simulink model "single_phase_ttype_inverter"  (R2026a)
settings: Solver=ode23tb  StopTime=simlength  FixedStep=tc  MaxStep=glb_time.tc
values from neighbouring files (symbols this model uses):
  afe_ctrl = param.afe.ctrl    [init_model.m]
  afe_pwm_phase_shift_mod1 = param.afe.behav.pwm_phase_shift_mod1    [init_model.m]
  DThs_init = param.thermal.DThs_init    [init_model.m]
  filters = param.ctrl.filters    [init_model.m]
  frt_data = param.frt.data    [init_model.m]
  glb_time = param.glb_time    [init_model.m]
  grid_emu = param.grid.emu    [init_model.m]
  kepsilon = param.spinv.kepsilon    [init_model.m]
  kp_align = param.ctrl.kp_align    [init_model.m]
  lim_down_align = param.ctrl.lim_down_align    [init_model.m]
  lim_up_align = param.ctrl.lim_up_align    [init_model.m]
  mavarage_filter_frequency_base_order = param.ctrl.mavarage_filter_frequency_base_order    [init_model.m]
  omega_set = param.spinv.omega_set    [init_model.m]
  single_phase_inverter_ctrl = param.spinv.ctrl    [init_model.m]
  Tambient = param.thermal.Tambient    [init_model.m]
  time_aux_power_supply_fault = param.sim.time_aux_power_supply_fault    [init_model.m]
  time_step_ref_1 = param.spinv.ref.time_step_ref_1    [init_model.m]
  time_step_ref_2 = param.spinv.ref.time_step_ref_2    [init_model.m]
  time_step_ref_3 = param.spinv.ref.time_step_ref_3    [init_model.m]
undefined symbols (not defined in the file or in its folder): delta_fht1, hwdata, ki_align, Ld_fht1, magnitude, omega_fht1, ts_inv, Vac_FS, Vdc_nom, Xbez
libraries: fl_lib x61, nesl_utility x39, moving_average_filter x11, moving_average_filter_cc x8, discrete_time_low_pass_filter x4, sl_discontinuities x3, single_phase_transformer_lib x3, linear_double_integrator_observer_ccaller x2, phase_shift_filter_ccaller x2, threephase_inductor_lib x1, dclink_for_two_levels x1, three_phase_pwm_modulator x1
(part 7 of 9)

== system single_phase_ttype_inverter/single_phase_inverter/single phase inverter control/single_phase_inverter_ctrl/phase generator/dq_pll_ccaller/first_harmonic_tracker3 ==
  u : Inport
  Bus Selector : BusSelector  OutputSignals=output_pu_hat
  Constant : Constant  Value=glb_time.ts_inv
  Constant1 : Constant  Value=4
  Constant2 : Constant  Value=afe_ctrl.fht_grid.omega_fht
  Constant3 : Constant  Value=afe_ctrl.fht_grid.delta_fht
  Constant4 : Constant  Value=afe_ctrl.fht_grid.Ld_fht(1)
  Constant5 : Constant  Value=afe_ctrl.fht_grid.Ld_fht(2)
  Data Type Conversion{1..2,6..9} (6 alike) : DataTypeConversion  OutDataTypeStr=single  SaturateOnIntegerOverflow=off  RndMeth=Floor
  Data Type Conversion3 : DataTypeConversion  OutDataTypeStr=uint8  SaturateOnIntegerOverflow=off  RndMeth=Floor
  Data Type Conversion4 : DataTypeConversion  OutDataTypeStr=double  SaturateOnIntegerOverflow=off  RndMeth=Floor
  Data Type Conversion5 : DataTypeConversion  OutDataTypeStr=uint8  SaturateOnIntegerOverflow=off  RndMeth=Floor
  Step : Step  Time=0.0125  InitialValue=1  FinalValue=0
  first_harmonic_tracker : CCaller  FunctionName=first_harmonic_tracker_process_simulink  PortSpecificationStruct="%)30     .    B \\   8    (     @         %    \"     D    !     0         %  0 \"0    $    _    07)G3F%M90  4&]R=$YA;64 4V-O<&4     26YD97@     5'EP90      4VEZ90      27-';&]B86P   X    P    !@    @    $          4    (     0    ,    !         !   P!O=70 #@   #     &    \"     0         !0    @    !     P    $         $  # &]U=  .    .     8    (    !          %    \"     $    &     0         0  ...(+4988 chars)"
  u_hat : Outport
  wires:
  Data Type Conversion4/1 -> u_hat/1
  Data Type Conversion3/1 -> first_harmonic_tracker/1
  Data Type Conversion1/1 -> first_harmonic_tracker/3
  Data Type Conversion2/1 -> first_harmonic_tracker/2
  first_harmonic_tracker/1 -> Bus Selector/1
  Bus Selector/1 -> Data Type Conversion4/1  "<output_pu_hat>"
  Step/1 -> Data Type Conversion3/1
  u/1 -> Data Type Conversion2/1
  Constant/1 -> Data Type Conversion1/1
  Constant1/1 -> Data Type Conversion5/1
  Data Type Conversion5/1 -> first_harmonic_tracker/8
  Constant2/1 -> Data Type Conversion6/1
  Data Type Conversion6/1 -> first_harmonic_tracker/4
  Constant3/1 -> Data Type Conversion7/1
  Data Type Conversion7/1 -> first_harmonic_tracker/5
  Constant4/1 -> Data Type Conversion8/1
  Data Type Conversion8/1 -> first_harmonic_tracker/6
  Constant5/1 -> Data Type Conversion9/1
  Data Type Conversion9/1 -> first_harmonic_tracker/7

== system single_phase_ttype_inverter/single_phase_inverter/single phase inverter control/single_phase_inverter_ctrl/phase_compensation_1/alignment_eval_afe1/pi ==
  u_ref : Inport
  u : Inport  Port=2
  1/Ti : Gain  Gain=kp  SaturateOnIntegerOverflow=on  OutDataTypeStr=Inherit: Same as input  ParamDataTypeStr=Inherit: Same as input
  Saturation : Saturate  UpperLimit=lim_up  LowerLimit=lim_down
  Sum1 : Sum  Inputs=+++  SaturateOnIntegerOverflow=on
  Sum2 : Sum  Inputs=-+  SaturateOnIntegerOverflow=on
  Sum3 : Sum  Inputs=-+  SaturateOnIntegerOverflow=on
  Unit Delay4 : UnitDelay  SampleTime=-1
  kp : Gain  Gain=ki  SaturateOnIntegerOverflow=on  OutDataTypeStr=Inherit: Same as input  ParamDataTypeStr=Inherit: Same as input
  y : Outport
  wires:
  1/Ti/1 -> Sum1/1, Sum3/1
  kp/1 -> Sum1/2
  Sum3/1 -> Unit Delay4/1
  Unit Delay4/1 -> Sum1/3
  u_ref/1 -> Sum2/2
  u/1 -> Sum2/1
  Sum2/1 -> kp/1, 1/Ti/1
  Sum1/1 -> Saturation/1
  Saturation/1 -> Sum3/2, y/1

== system single_phase_ttype_inverter/single_phase_inverter/single phase inverter control/single_phase_inverter_ctrl/single_phase_current_control/dqpi_current_controller/alphabeta2dq ==
  alpha : Inport
  beta : Inport  Port=2
  MATLAB Function : MATLAB Function  TreatAsAtomicUnit=on
  "d " : Outport  VectorParamsAs1DForOutWhenUnconnected=off
  "q " : Outport  Port=2  VectorParamsAs1DForOutWhenUnconnected=off
  wires:
  alpha/1 -> MATLAB Function/1(alpha)
  beta/1 -> MATLAB Function/2(beta)
  MATLAB Function/1(d) -> "d "/1
  MATLAB Function/2(q) -> "q "/1
  [phase] -> MATLAB Function/3(phase)

== system single_phase_ttype_inverter/single_phase_inverter/single phase inverter control/single_phase_inverter_ctrl/single_phase_current_control/dqpi_current_controller/dq2alphabeta ==
  d : Inport
  q : Inport  Port=2
  MATLAB Function : MATLAB Function  TreatAsAtomicUnit=on
  alpha : Outport  VectorParamsAs1DForOutWhenUnconnected=off
  wires:
  d/1 -> MATLAB Function/1(d)
  q/1 -> MATLAB Function/2(q)
  MATLAB Function/1(alpha) -> alpha/1
  [phase] -> MATLAB Function/3(phase)

== system single_phase_ttype_inverter/single_phase_inverter/single phase inverter control/single_phase_inverter_ctrl/single_phase_current_control/dqpi_current_controller/dq_vector_pi ==
  id_ref : Inport
  id : Inport  Port=2
  iq : Inport  Port=3
  iq_ref : Inport  Port=4
  dq_vector_pi : dq_vector_pi/dq_vector_pi  kp=single_phase_inverter_ctrl.kp_inv  ki=single_phase_inverter_ctrl.ki_inv  ts=glb_time.ts_inv  lim_ctrl_out=1  CTRPIFF_CLIP_RELEASE=1e-3
  ud_ctrl : Outport
  uq_ctrl : Outport  Port=2
  wires:
  id_ref/1 -> dq_vector_pi/1  "id_ref"
  iq_ref/1 -> dq_vector_pi/3  "iq_ref"
  dq_vector_pi/1 -> ud_ctrl/1  "ud_ctrl"
  iq/1 -> dq_vector_pi/4  "iq"
  id/1 -> dq_vector_pi/2  "id"
  dq_vector_pi/2 -> uq_ctrl/1  "uq_ctrl"
  [dclink_voltage_pu] -> dq_vector_pi/5

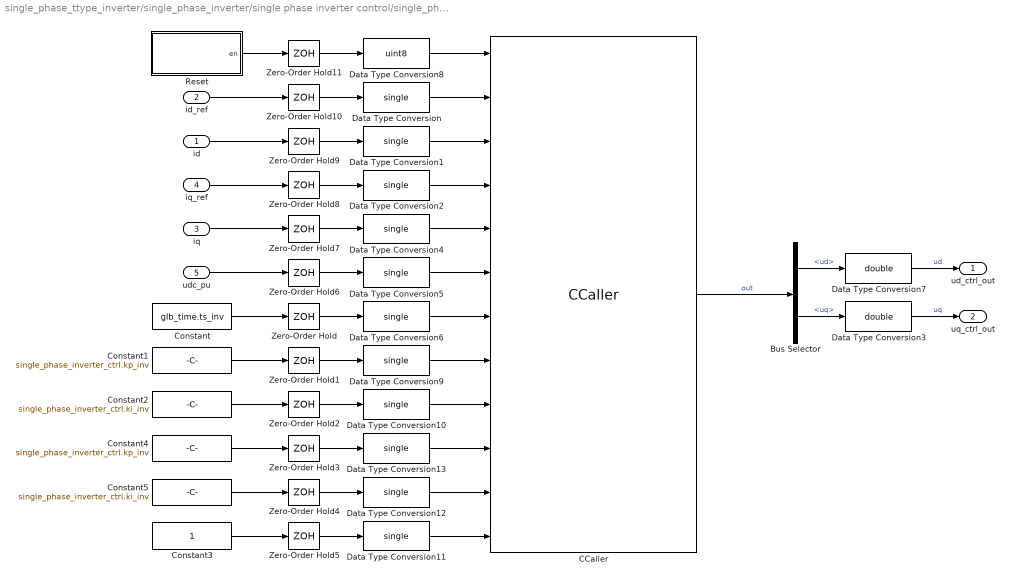
== system single_phase_ttype_inverter/single_phase_inverter/single phase inverter control/single_phase_inverter_ctrl/single_phase_current_control/dqpi_current_controller/dq_vector_pi_ccaller ==
  id : Inport
  id_ref : Inport  Port=2
  iq : Inport  Port=3
  iq_ref : Inport  Port=4
  udc_pu : Inport  Port=5
  Bus Selector : BusSelector  OutputSignals=ud,uq
  CCaller : CCaller  FunctionName=dqvector_pi_process_simulink  PortSpecificationStruct="%)30     .    ,!8   8    (     @         %    \"     T    !     0         %  0 \"0    $    _    07)G3F%M90  4&]R=$YA;64 4V-O<&4     26YD97@     5'EP90      4VEZ90      27-';&]B86P   X    P    !@    @    $          4    (     0    ,    !         !   P!O=70 #@   #     &    \"     0         !0    @    !     P    $         $  # &]U=  .    .     8    (    !          %    \"     $    &     0         0   ...(+7280 chars)"
  Constant : Constant  Value=glb_time.ts_inv
  Constant1 : Constant  Value=single_phase_inverter_ctrl.kp_inv
  Constant2 : Constant  Value=single_phase_inverter_ctrl.ki_inv
  Constant3 : Constant
  Constant4 : Constant  Value=single_phase_inverter_ctrl.kp_inv
  Constant5 : Constant  Value=single_phase_inverter_ctrl.ki_inv
  Data Type Conversion{,1..2,4..6,9..13} (11 alike) : DataTypeConversion  OutDataTypeStr=single  SaturateOnIntegerOverflow=off  RndMeth=Floor
  Data Type Conversion3 : DataTypeConversion  OutDataTypeStr=double  SaturateOnIntegerOverflow=off  RndMeth=Floor
  Data Type Conversion7 : DataTypeConversion  OutDataTypeStr=double  SaturateOnIntegerOverflow=off  RndMeth=Floor
  Data Type Conversion8 : DataTypeConversion  OutDataTypeStr=uint8  SaturateOnIntegerOverflow=off  RndMeth=Floor
  Reset : Subsystem
  Zero-Order Hold{,1..11} (12 alike) : ZeroOrderHold  SampleTime=-1
  ud_ctrl_out : Outport
  uq_ctrl_out : Outport  Port=2
  wires:
  Data Type Conversion5/1 -> CCaller/6
  Data Type Conversion/1 -> CCaller/2
  CCaller/1 -> Bus Selector/1  "out"
  Data Type Conversion1/1 -> CCaller/3
  Data Type Conversion4/1 -> CCaller/5
  Data Type Conversion2/1 -> CCaller/4
  Data Type Conversion6/1 -> CCaller/7
  Bus Selector/2 -> Data Type Conversion3/1  "<uq>"
  Bus Selector/1 -> Data Type Conversion7/1  "<ud>"
  Data Type Conversion7/1 -> ud_ctrl_out/1  "ud"
  Data Type Conversion3/1 -> uq_ctrl_out/1  "uq"
  Data Type Conversion8/1 -> CCaller/1
  Data Type Conversion9/1 -> CCaller/8
  Data Type Conversion10/1 -> CCaller/9
  Data Type Conversion11/1 -> CCaller/12
  Data Type Conversion13/1 -> CCaller/10
  Data Type Conversion12/1 -> CCaller/11
  Constant3/1 -> Zero-Order Hold5/1
  Constant5/1 -> Zero-Order Hold4/1
  Constant4/1 -> Zero-Order Hold3/1
  Constant2/1 -> Zero-Order Hold2/1
  Constant1/1 -> Zero-Order Hold1/1
  Constant/1 -> Zero-Order Hold/1
  udc_pu/1 -> Zero-Order Hold6/1
  iq/1 -> Zero-Order Hold7/1
  iq_ref/1 -> Zero-Order Hold8/1
  Reset/1(en) -> Zero-Order Hold11/1
  id_ref/1 -> Zero-Order Hold10/1
  id/1 -> Zero-Order Hold9/1
  Zero-Order Hold/1 -> Data Type Conversion6/1
  Zero-Order Hold1/1 -> Data Type Conversion9/1
  Zero-Order Hold2/1 -> Data Type Conversion10/1
  Zero-Order Hold3/1 -> Data Type Conversion13/1
  Zero-Order Hold4/1 -> Data Type Conversion12/1
  Zero-Order Hold5/1 -> Data Type Conversion11/1
  Zero-Order Hold6/1 -> Data Type Conversion5/1
  Zero-Order Hold7/1 -> Data Type Conversion4/1
  Zero-Order Hold8/1 -> Data Type Conversion2/1
  Zero-Order Hold9/1 -> Data Type Conversion1/1
  Zero-Order Hold10/1 -> Data Type Conversion/1
  Zero-Order Hold11/1 -> Data Type Conversion8/1

== system single_phase_ttype_inverter/single_phase_inverter/single phase inverter control/single_phase_inverter_ctrl/single_phase_current_control/dqpi_current_controller/i2alphabeta ==
  i_alpha : Inport
  Variant Source2 : VariantSource  VariantControls="{use_single_phase_inverter_based_FHT == 1, use_single_phase_inverter_based_SOGI  == 1, use_single_phase_inverter_based_PHSH  == 1, use_single_phase_inverter_based_SOGI_ccaller  == 1, use_single_phase_inverter_based_PHSH_ccaller  == 1}"
  Variant Source3 : VariantSource  VariantControls="{use_single_phase_inverter_based_FHT == 1, use_single_phase_inverter_based_SOGI  == 1, use_single_phase_inverter_based_PHSH  == 1, use_single_phase_inverter_based_SOGI_ccaller  == 1, use_single_phase_inverter_based_PHSH_ccaller  == 1}"
  first_harmonic_tracker : Subsystem
  phase_shift_method : Subsystem
  phase_shift_method_ccaller : Subsystem
  sogi : Subsystem
  sogi_ccaller : Subsystem
  i_alpha_out : Outport
  i_beta_out : Outport  Port=2
  wires:
  i_alpha/1 -> phase_shift_method_ccaller/1(i_alpha), sogi_ccaller/1(input), phase_shift_method/1(i_alpha), sogi/1(u), first_harmonic_tracker/1(u)
  [i_alpha_phsh] -> Variant Source2/3
  [i_beta_sogi] -> Variant Source3/2
  [i_alpha_phsh_cc] -> Variant Source2/5
  first_harmonic_tracker/2(beta) -> [i_beta_fht]  "i_beta_fht"
  phase_shift_method/2(i_beta_phase_shift_m) -> [i_beta_phsh]  "i_beta_phsh"
  phase_shift_method/1(i_alpha_phase_shift_m) -> [i_alpha_phsh]  "i_alpha_phsh"
  [i_alpha_sogi] -> Variant Source2/2
  phase_shift_method_ccaller/1(i_alpha_phase_shift_m) -> [i_alpha_phsh_cc]  "i_alpha_phsh_cc"
  [i_beta_phsh_cc] -> Variant Source3/5
  [i_alpha_fht] -> Variant Source2/1
  [i_beta_phsh] -> Variant Source3/3
  sogi_ccaller/1(alpha) -> [i_alpha_sogi_cc]  "i_alpha_sogi_cc"
  [i_beta_sogi_cc] -> Variant Source3/4
  sogi/1(ualpha) -> [i_alpha_sogi]  "i_alpha_sogi"
  sogi/2(ubeta) -> [i_beta_sogi]  "i_beta_sogi"
  phase_shift_method_ccaller/2(i_beta_phase_shift_m) -> [i_beta_phsh_cc]  "i_beta_phsh_cc"
  sogi_ccaller/2(beta) -> [i_beta_sogi_cc]  "i_beta_sogi_cc"
  Variant Source2/1 -> i_alpha_out/1  "i_alpha"
  first_harmonic_tracker/1(alpha) -> [i_alpha_fht]  "i_alpha_fht"
  [i_alpha_sogi_cc] -> Variant Source2/4
  [i_beta_fht] -> Variant Source3/1
  Variant Source3/1 -> i_beta_out/1  "i_beta"

== system single_phase_ttype_inverter/single_phase_inverter/single phase inverter control/single_phase_inverter_ctrl/single_phase_current_control/rpi_current_controller/Reset ==
  Step : Step  Time=0.05  InitialValue=1  FinalValue=0
  en : Outport
  wires:
  Step/1 -> en/1

== system single_phase_ttype_inverter/single_phase_inverter/single phase inverter control/single_phase_inverter_ctrl/sistem_identification/open loop u//f/dq2alphabeta ==
  Constant1 : Constant  Value=0
  Data Store Read : DataStoreRead  DataStoreName=u_test  IndexOptions=Index vector (dialog)  Indices=1  OutputSizes=1
  MATLAB Function : MATLAB Function  TreatAsAtomicUnit=on
  alpha : Outport  VectorParamsAs1DForOutWhenUnconnected=off
  wires:
  [phase] -> MATLAB Function/3(phase)
  MATLAB Function/1(alpha) -> alpha/1
  Data Store Read/1 -> MATLAB Function/1(d)
  Constant1/1 -> MATLAB Function/2(q)

== system single_phase_ttype_inverter/single_phase_inverter/single phase inverter control/single_phase_inverter_ctrl/sistem_identification/open loop u//f/first_harmonic_tracker ==
  u : Inport
  Bus Selector : BusSelector  OutputSignals=output_pu_hat,output_pu_hat_dot
  Constant : Constant  Value=ts_inv
  Constant1 : Constant  Value=8
  Constant2 : Constant  Value=omega_fht1
  Constant3 : Constant  Value=delta_fht1
  Constant4 : Constant  Value=Ld_fht1(1)
  Constant5 : Constant  Value=Ld_fht1(2)
  Data Type Conversion{1..2,6..9} (6 alike) : DataTypeConversion  OutDataTypeStr=single  SaturateOnIntegerOverflow=off  RndMeth=Floor
  Data Type Conversion10 : DataTypeConversion  OutDataTypeStr=double  SaturateOnIntegerOverflow=off  RndMeth=Floor
  Data Type Conversion3 : DataTypeConversion  OutDataTypeStr=uint8  SaturateOnIntegerOverflow=off  RndMeth=Floor
  Data Type Conversion4 : DataTypeConversion  OutDataTypeStr=double  SaturateOnIntegerOverflow=off  RndMeth=Floor
  Data Type Conversion5 : DataTypeConversion  OutDataTypeStr=uint8  SaturateOnIntegerOverflow=off  RndMeth=Floor
  Gain : Gain  Gain=-1/omega_fht1
  Step : Step  Time=0.0125  InitialValue=1  FinalValue=0
  first_harmonic_tracker : CCaller  FunctionName=first_harmonic_tracker_process_simulink  PortSpecificationStruct="%)30     .    B \\   8    (     @         %    \"     D    !     0         %  0 \"0    $    _    07)G3F%M90  4&]R=$YA;64 4V-O<&4     26YD97@     5'EP90      4VEZ90      27-';&]B86P   X    P    !@    @    $          4    (     0    ,    !         !   P!O=70 #@   #     &    \"     0         !0    @    !     P    $         $  # &]U=  .    .     8    (    !          %    \"     $    &     0         0  ...(+4988 chars)"
  alpha : Outport
  beta : Outport  Port=2
  wires:
  Data Type Conversion4/1 -> alpha/1
  Data Type Conversion3/1 -> first_harmonic_tracker/1
  Data Type Conversion1/1 -> first_harmonic_tracker/3
  Data Type Conversion2/1 -> first_harmonic_tracker/2
  first_harmonic_tracker/1 -> Bus Selector/1
  Bus Selector/1 -> Data Type Conversion4/1  "<output_pu_hat>"
  Step/1 -> Data Type Conversion3/1
  u/1 -> Data Type Conversion2/1
  Constant/1 -> Data Type Conversion1/1
  Constant1/1 -> Data Type Conversion5/1
  Data Type Conversion5/1 -> first_harmonic_tracker/8
  Constant2/1 -> Data Type Conversion6/1
  Data Type Conversion6/1 -> first_harmonic_tracker/4
  Constant3/1 -> Data Type Conversion7/1
  Data Type Conversion7/1 -> first_harmonic_tracker/5
  Constant4/1 -> Data Type Conversion8/1
  Data Type Conversion8/1 -> first_harmonic_tracker/6
  Constant5/1 -> Data Type Conversion9/1
  Data Type Conversion9/1 -> first_harmonic_tracker/7
  Bus Selector/2 -> Data Type Conversion10/1  "<output_pu_hat_dot>"
  Data Type Conversion10/1 -> Gain/1
  Gain/1 -> beta/1

== system single_phase_ttype_inverter/single_phase_inverter/single phase inverter control/single_phase_inverter_ctrl/sistem_identification/open loop u//f/module ==
  i_alpha : Inport
  i_beta : Inport  Port=2
  Sqrt : Sqrt
  Square : Math  Operator=square
  Square1 : Math  Operator=square
  Sum : Sum  Inputs=|++
  i : Outport
  wires:
  i_beta/1 -> Square1/1
  i_alpha/1 -> Square/1
  Square/1 -> Sum/1
  Sum/1 -> Sqrt/1
  Square1/1 -> Sum/2
  Sqrt/1 -> i/1  "i"

== system single_phase_ttype_inverter/single_phase_inverter/single phase inverter control/single_phase_inverter_ctrl/sistem_identification/open loop u//f/sogi_ccaller ==
  input : Inport
  Bus Selector : BusSelector  OutputSignals=sogi_flt_output_alpha,sogi_flt_output_beta
  CCaller : CCaller  FunctionName=sogi_flt_process_simulink  PortSpecificationStruct="%)30     .    . P   8    (     @         %    \"     <    !     0         %  0 \"0    $    _    07)G3F%M90  4&]R=$YA;64 4V-O<&4     26YD97@     5'EP90      4VEZ90      27-';&]B86P   X    P    !@    @    $          4    (     0    ,    !         !   P!O=70 #@   #     &    \"     0         !0    @    !     P    $         $  # &]U=  .    .     8    (    !          %    \"     $    &     0         0   ...(+3829 chars)"
  Constant1 : Constant  Value=ts_inv
  Constant2 : Constant  Value=omega_set
  Constant3 : Constant  Value=kepsilon
  Constant4 : Constant  Value=0
  Data Type Conversion{1..2,4,6} (4 alike) : DataTypeConversion  OutDataTypeStr=single  SaturateOnIntegerOverflow=off  RndMeth=Floor
  Data Type Conversion3 : DataTypeConversion  OutDataTypeStr=uint8  SaturateOnIntegerOverflow=off  RndMeth=Floor
  Data Type Conversion5 : DataTypeConversion  OutDataTypeStr=double  SaturateOnIntegerOverflow=off  RndMeth=Floor
  Data Type Conversion7 : DataTypeConversion  OutDataTypeStr=double  SaturateOnIntegerOverflow=off  RndMeth=Floor
  Data Type Conversion8 : DataTypeConversion  OutDataTypeStr=uint8  SaturateOnIntegerOverflow=off  RndMeth=Floor
  Reset : Subsystem
  Zero-Order Hold{1..6} (6 alike) : ZeroOrderHold  SampleTime=-1
  alpha : Outport
  beta : Outport  Port=2
  wires:
  Zero-Order Hold6/1 -> Data Type Conversion4/1
  Data Type Conversion7/1 -> alpha/1
  Data Type Conversion4/1 -> CCaller/1
  Bus Selector/1 -> Data Type Conversion7/1  "<sogi_flt_output_alpha>"
  CCaller/1 -> Bus Selector/1
  Constant4/1 -> Zero-Order Hold5/1
  Zero-Order Hold5/1 -> Data Type Conversion3/1
  Constant2/1 -> Zero-Order Hold1/1
  Zero-Order Hold1/1 -> Data Type Conversion2/1
  Zero-Order Hold2/1 -> Data Type Conversion1/1
  Constant1/1 -> Zero-Order Hold2/1
  Reset/1(en) -> Zero-Order Hold4/1
  Zero-Order Hold4/1 -> Data Type Conversion8/1
  input/1 -> Zero-Order Hold6/1
  Bus Selector/2 -> Data Type Conversion5/1  "<sogi_flt_output_beta>"
  Data Type Conversion5/1 -> beta/1
  Data Type Conversion3/1 -> CCaller/6
  Data Type Conversion8/1 -> CCaller/5
  Data Type Conversion2/1 -> CCaller/3
  Data Type Conversion1/1 -> CCaller/2
  Data Type Conversion6/1 -> CCaller/4
  Zero-Order Hold3/1 -> Data Type Conversion6/1
  Constant3/1 -> Zero-Order Hold3/1

== system single_phase_ttype_inverter/afe/AFE_control/afe_control/current_ctrl/inner_current_ctrl/anti_wind_up_ff/anti_wind_up ==
  alpha : Inport
  beta : Inport  Port=2
  Saturation : Saturate  UpperLimit=10  LowerLimit=1
  Sqrt : Sqrt
  Square : Math  Operator=square
  Square1 : Math  Operator=square
  Sum : Sum  Inputs=|++
  scaling : Outport
  wires:
  alpha/1 -> Square/1
  Sum/1 -> Sqrt/1
  beta/1 -> Square1/1
  Square/1 -> Sum/1
  Square1/1 -> Sum/2
  Sqrt/1 -> Saturation/1
  Saturation/1 -> scaling/1

== system single_phase_ttype_inverter/afe/AFE_control/afe_control/grid_voltage_phase_lock_loops/DDSRF-PLL/pll_stageA/filter_and_transformation ==
  ug_a : Inport
  ug_b : Inport  Port=2
  ug_c : Inport  Port=3
  abc2alphabeta : MATLAB Function  TreatAsAtomicUnit=on
  first_harmonic_tracker : Scope  NumInputPorts=3
      settings: ActiveDisplayYMinimum=-1.2482939809560776  ActiveDisplayYMaximum=1.2484282106161118  DataLoggingVariableName=ScopeData3
  first_harmonic_tracker_phase_u : Subsystem
  first_harmonic_tracker_phase_v : Subsystem
  first_harmonic_tracker_phase_w : Subsystem
  ug_alpha : Outport  VectorParamsAs1DForOutWhenUnconnected=off
  ug_beta : Outport  Port=2  VectorParamsAs1DForOutWhenUnconnected=off
  wires:
  abc2alphabeta/1(alpha) -> ug_alpha/1  "u_grid_alpha"
  abc2alphabeta/2(beta) -> ug_beta/1  "u_grid_beta"
  first_harmonic_tracker_phase_u/1(u_hat) -> first_harmonic_tracker/1, abc2alphabeta/1(a)  "tracker_phase_u"
  first_harmonic_tracker_phase_w/1(u_hat) -> first_harmonic_tracker/3, abc2alphabeta/3(c)  "tracker_phase_w"
  first_harmonic_tracker_phase_v/1(u_hat) -> first_harmonic_tracker/2, abc2alphabeta/2(b)  "tracker_phase_v"
  ug_a/1 -> first_harmonic_tracker_phase_u/1(u)
  ug_b/1 -> first_harmonic_tracker_phase_v/1(u)
  ug_c/1 -> first_harmonic_tracker_phase_w/1(u)

== system single_phase_ttype_inverter/afe/AFE_control/afe_control/grid_voltage_phase_lock_loops/DDSRF-PLL/pll_stageA/sequences ==
  u_grid_alpha : Inport
  u_grid_beta : Inport  Port=2
  phase_angle : Inport  Port=3
  ddsrf : Subsystem
  u_grid_pos_xi : Outport
  u_grid_pos_eta : Outport  Port=2
  wires:
  phase_angle/1 -> ddsrf/3(phase_angle)  "phase_angle"
  u_grid_beta/1 -> ddsrf/2(u_grid_beta)  "u_grid_beta"
  u_grid_alpha/1 -> ddsrf/1(u_grid_alpha)  "u_grid_alpha"
  ddsrf/4(u_grid_neg_eta) -> u_grid_pos_eta/1  "u_grid_pos_eta"
  ddsrf/3(u_grid_neg_xi) -> u_grid_pos_xi/1  "u_grid_pos_xi"

== system single_phase_ttype_inverter/afe/AFE_control/afe_control/grid_voltage_phase_lock_loops/DDSRF-PLL/pll_stageB/double_integrator_observer ==
  phase : Inport
  Gain : Gain  Gain=afe_ctrl.di_obs.Ldso  Multiplication=Matrix(K*u)
  Gain1 : Gain  Gain=afe_ctrl.di_obs.Adso  Multiplication=Matrix(K*u)
  Gain2 : Gain  Gain=afe_ctrl.di_obs.Cso  Multiplication=Matrix(K*u)
  Selector : Selector  InputPortWidth=2  IndexOptions=Index vector (dialog)  Indices=2  OutputSizes=1
  Sum : Sum  Inputs=-+|
  Sum1 : Sum  Inputs=|++
  Unit Delay : UnitDelay  SampleTime=-1
  bounder1 : MATLAB Function  TreatAsAtomicUnit=on
  bounder2 : MATLAB Function  TreatAsAtomicUnit=on
  omega_hat : Outport
  wires:
  Gain/1 -> Sum1/1
  Selector/1 -> omega_hat/1
  Gain2/1 -> bounder2/1(u)  "theta_hat"
  Gain1/1 -> Sum1/2
  Sum1/1 -> Unit Delay/1
  Sum/1 -> bounder1/1(u)  "e"
  Unit Delay/1 -> Gain1/1, Selector/1, Gain2/1
  phase/1 -> Sum/2  "phase"
  bounder1/1(y) -> Gain/1  "e_bounded"
  bounder2/1(y) -> Sum/1  "theta_hat_bounded"

== system single_phase_ttype_inverter/afe/AFE_control/afe_control/grid_voltage_phase_lock_loops/FHT-PLL/pll_stageA/filter_and_transformation ==
  ug_a : Inport
  ug_b : Inport  Port=2
  ug_c : Inport  Port=3
  Bus Creator : BusCreator  Inputs=2
  Bus Creator1 : BusCreator  Inputs=3
  Bus Creator2 : BusCreator  Inputs=2
  Bus Creator3 : BusCreator  Inputs=3
  Bus Creator4 : BusCreator  Inputs=3
  FHTalpha : Subsystem
  FHTbeta : Subsystem
  FHTdqPLL : Scope  NumInputPorts=2
      settings: ActiveDisplayYMinimum=-1.5258214459194912  ActiveDisplayYMaximum=1.5258228058860459  DataLoggingVariableName=ScopeData12
  Gain : Gain  Gain=-1/2
  Gain1 : Gain  Gain=-1/2
  Sum : Sum  Inputs=|++
  Sum1 : Sum  Inputs=-+|
  To Workspace1 : ToWorkspace  VariableName=ugd_alpha_sim  SampleTime=-1
      settings: MaxDataPoints=glb_time.Ns_afe
  To Workspace2 : ToWorkspace  VariableName=ugd_beta_sim  SampleTime=-1
      settings: MaxDataPoints=glb_time.Ns_afe
  To Workspace3 : ToWorkspace  VariableName=u_fht_alpha_sim  SampleTime=-1
      settings: MaxDataPoints=glb_time.Ns_afe
  To Workspace4 : ToWorkspace  VariableName=v_fht_alpha_sim  SampleTime=-1
      settings: MaxDataPoints=glb_time.Ns_afe
  To Workspace5 : ToWorkspace  VariableName=u_fhtsr_alpha_sim  SampleTime=-1
      settings: MaxDataPoints=glb_time.Ns_afe
  To Workspace6 : ToWorkspace  VariableName=u_fhtsr_beta_sim  SampleTime=-1
      settings: MaxDataPoints=glb_time.Ns_afe
  To Workspace7 : ToWorkspace  VariableName=u_fht_beta_sim  SampleTime=-1
      settings: MaxDataPoints=glb_time.Ns_afe
  To Workspace8 : ToWorkspace  VariableName=v_fht_beta_sim  SampleTime=-1
      settings: MaxDataPoints=glb_time.Ns_afe
  To Workspace9 : ToWorkspace  VariableName=ugd_abc_grid_sim  SampleTime=-1
      settings: MaxDataPoints=glb_time.Ns_afe
  abc2alphabeta : MATLAB Function  TreatAsAtomicUnit=on
  grid_voltages : Scope  NumInputPorts=3
      settings: ActiveDisplayYMinimum=-1.3618303835391998  ActiveDisplayYMaximum=1.3331545889377594  DataLoggingVariableName=ScopeData13
  ug_alpha : Outport  VectorParamsAs1DForOutWhenUnconnected=off
  ug_beta : Outport  Port=2  VectorParamsAs1DForOutWhenUnconnected=off
  wires:
  ug_b/1 -> Bus Creator3/2, grid_voltages/2, abc2alphabeta/2(b)  "ugd_b"
  ug_c/1 -> Bus Creator3/3, grid_voltages/3, abc2alphabeta/3(c)  "ugd_c"
  ug_a/1 -> Bus Creator3/1, grid_voltages/1, abc2alphabeta/1(a)  "ugd_a"
  abc2alphabeta/1(alpha) -> To Workspace1/1, FHTalpha/1(u), Bus Creator4/1  "u_grid_alpha"
  abc2alphabeta/2(beta) -> FHTbeta/1(u), To Workspace2/1, Bus Creator1/1  "u_grid_beta"
  FHTalpha/1(ud_hat) -> To Workspace3/1, Bus Creator/1, Sum/1  "u_fht_alpha"
  Sum/1 -> Gain/1
  FHTbeta/1(ud_hat) -> Sum1/2, To Workspace7/1, Bus Creator2/1  "u_fht_beta"
  Sum1/1 -> Gain1/1
  Gain1/1 -> Bus Creator1/3, To Workspace6/1, ug_beta/1  "u_fhtsr_beta"
  Gain/1 -> Bus Creator4/3, To Workspace5/1, ug_alpha/1  "u_fhtsr_alpha"
  FHTbeta/2(uq_hat) -> Sum/2, To Workspace8/1, Bus Creator2/2  "v_fht_beta"
  FHTalpha/2(uq_hat) -> Sum1/1, To Workspace4/1, Bus Creator/2  "v_fht_alpha"
  Bus Creator1/1 -> FHTdqPLL/2
  Bus Creator4/1 -> FHTdqPLL/1
  Bus Creator/1 -> Bus Creator4/2  "FHTalpha"
  Bus Creator2/1 -> Bus Creator1/2  "FHTbeta"
  Bus Creator3/1 -> To Workspace9/1

== system single_phase_ttype_inverter/afe/AFE_control/afe_control/grid_voltage_phase_lock_loops/FHT-PLL/pll_stageA/sequences ==
  u_grid_alpha : Inport
  u_grid_beta : Inport  Port=2
  phase_angle : Inport  Port=3
  alphabeta2xieta : MATLAB Function  TreatAsAtomicUnit=on
  u_grid_xi : Outport
  u_grid_eta : Outport  Port=2
  wires:
  alphabeta2xieta/1(xi) -> u_grid_xi/1  "u_grid_xi"
  alphabeta2xieta/2(eta) -> u_grid_eta/1  "u_grid_eta"
  u_grid_alpha/1 -> alphabeta2xieta/1(alpha)  "u_grid_alpha"
  u_grid_beta/1 -> alphabeta2xieta/2(beta)  "u_grid_beta"
  phase_angle/1 -> alphabeta2xieta/3(gamma)  "phase_angle"

== system single_phase_ttype_inverter/afe/AFE_control/afe_control/grid_voltage_phase_lock_loops/FHT-PLL/pll_stageB/double_integrator_observer ==
  theta : Inport
  Gain : Gain  Gain=afe_ctrl.di_obs.Ldso  Multiplication=Matrix(K*u)
  Gain1 : Gain  Gain=afe_ctrl.di_obs.Adso  Multiplication=Matrix(K*u)
  Gain2 : Gain  Gain=afe_ctrl.di_obs.Cso  Multiplication=Matrix(K*u)
  Selector : Selector  InputPortWidth=2  IndexOptions=Index vector (dialog)  Indices=2  OutputSizes=1
  Sum : Sum  Inputs=-+|
  Sum1 : Sum  Inputs=|++
  Unit Delay : UnitDelay  SampleTime=-1
  bounder1 : MATLAB Function  TreatAsAtomicUnit=on
  bounder2 : MATLAB Function  TreatAsAtomicUnit=on
  omega_hat : Outport
  wires:
  Gain/1 -> Sum1/1
  Selector/1 -> omega_hat/1
  Gain2/1 -> bounder2/1(u)  "theta_hat"
  Gain1/1 -> Sum1/2
  Sum1/1 -> Unit Delay/1
  Sum/1 -> bounder1/1(u)  "e"
  Unit Delay/1 -> Gain1/1, Selector/1, Gain2/1
  theta/1 -> Sum/2  "theta"
  bounder1/1(y) -> Gain/1
  bounder2/1(y) -> Sum/1  "theta_hat_bounded"

== system single_phase_ttype_inverter/afe/AFE_control/afe_control/grid_voltage_phase_lock_loops/dq_pll/pll_stageA/mormalization_and_transformation ==
  ug_a : Inport
  ug_b : Inport  Port=2
  ug_c : Inport  Port=3
  abc2alphabeta : MATLAB Function  TreatAsAtomicUnit=on
  ug_alpha : Outport  VectorParamsAs1DForOutWhenUnconnected=off
  ug_beta : Outport  Port=2  VectorParamsAs1DForOutWhenUnconnected=off
  wires:
  abc2alphabeta/2(beta) -> ug_beta/1  "u_grid_beta"
  abc2alphabeta/1(alpha) -> ug_alpha/1  "u_grid_alpha"
  ug_a/1 -> abc2alphabeta/1(a)
  ug_b/1 -> abc2alphabeta/2(b)
  ug_c/1 -> abc2alphabeta/3(c)

== system single_phase_ttype_inverter/afe/AFE_control/afe_control/grid_voltage_phase_lock_loops/dq_pll/pll_stageA/sequences ==
  u_grid_alpha : Inport
  u_grid_beta : Inport  Port=2
  gamma_grid : Inport  Port=3
  alphabeta2xieta : Subsystem
  u_grid_pos_xi : Outport
  u_grid_pos_eta : Outport  Port=2
  wires:
  alphabeta2xieta/1(xi) -> u_grid_pos_xi/1  "u_grid_pos_xi"
  alphabeta2xieta/2(eta) -> u_grid_pos_eta/1  "u_grid_pos_eta"
  u_grid_alpha/1 -> alphabeta2xieta/1(alpha)  "u_grid_alpha"
  u_grid_beta/1 -> alphabeta2xieta/2(beta)  "u_grid_beta"
  gamma_grid/1 -> alphabeta2xieta/3(gamma)  "phase_grid"
